simulink model "Evaluation_RL_SMC_Env"  (R2024b)
settings: Solver=VariableStepAuto  StartTime=0.0  StopTime=60  RelTol=1e-3
values from neighbouring files (symbols this model uses):
  D = [0; 0]    [K_vector_2.m]
undefined symbols (not defined in the file or in its folder): ref_seed
libraries: simulink x7, dspstat3 x4, rllib x2, slctrl_smc x1
settings Model: Creator=minhh  LastModifiedBy=minhh
settings DebuggingCC: SignalInfNanChecking=error

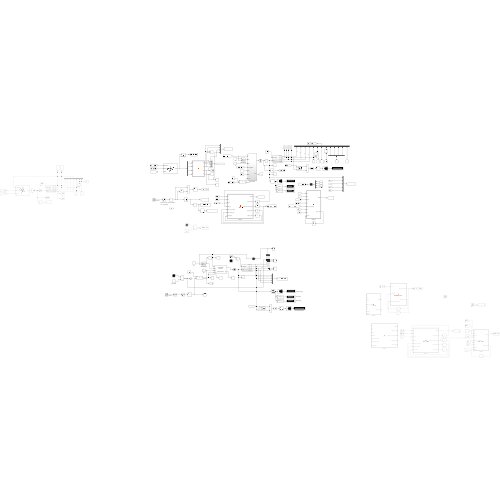
[thumbnail: Simulink's stored preview of the top-level diagram]
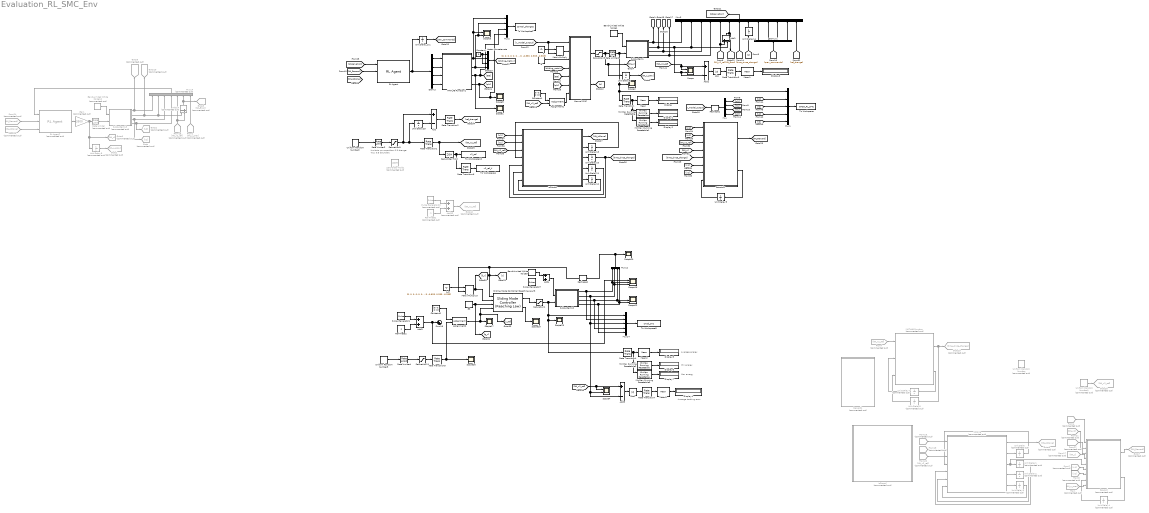
== system Evaluation_RL_SMC_Env ==
  note: Average energy
  note: Limits to no more than 0.3 change;
      | -0.2; 0.5 boundary
  note: Min energy
  note: Max energy
  note: Average tracking error
  A : Constant  Value=[0, 0, 0, 0; 0, 0, 0, 1; -4, 1, -0.5, 0.4; 0.833, -0.833, 0.333, -0.333]  VectorParams1D=off
  A_3 : Constant  Value=[0, 0, 0, 0; 0, 0, 0, 1; -4, 1, -0.5, 0.4; 0.833, -0.833, 0.333, -0.333]  VectorParams1D=off
  Abs : Abs  SaturateOnIntegerOverflow=off
  Abs1 : Abs  SaturateOnIntegerOverflow=off
  Add{,1..2,5} (4 alike) : Sum  Inputs=+-
  Add12 : Sum  Commented=on
  Add14 : Sum  Commented=on  Inputs=-+
  Add3 : Sum
  Add4 : Sum
  Assignment1 : Assignment  DiagnosticForDimensions=Warning  IndexOptions=Index vector (dialog)  Indices=2  OutputSizes=1
  Assignment2 : Assignment  DiagnosticForDimensions=Warning  IndexOptions=Index vector (dialog)  Indices=2  OutputSizes=1
  B : Constant  Value=[0; 0.004; 0; 0]
  B3 : Constant  Value=[0; 0.004; 0; 0]
  Band-Limited White Noise1 : simulink/Sources/Band-Limited White Noise  Cov=[200]  Ts=0.01  seed=23341
  Band-Limited White Noise12 : simulink/Sources/Band-Limited White Noise  Commented=on  Cov=[200]  Ts=0.01  seed=noise_seed
  Band-Limited White Noise9 : simulink/Sources/Band-Limited White Noise  Cov=[200]  Ts=0.01  seed=[23341]
  Constant : Constant  Value=0
  Constant1 : Constant  Value=[0; 0; 0; 0]  VectorParams1D=off
  Constant2 : Constant  Value=[0; 0; 0; 0]  VectorParams1D=off
  Demux : Demux
  Demux1 : Demux
  Display{,1..7} (8 alike) : Display
  From : From  Commented=on  GotoTag=NN_u_prev
  From1 : From  Commented=on  GotoTag=NN_u_prev
  From{7,15,20,22} (4 alike) : From  Commented=on  GotoTag=NN_x2_ref
  From17 : From  Commented=on  GotoTag=NN_u
  From18 : From  Commented=on  GotoTag=NN_x1
  From19 : From  Commented=on  GotoTag=NN_x2
  From2 : From  Commented=on  GotoTag=v1
  From21 : From  Commented=on  GotoTag=NN_x2
  From23 : From  Commented=on  GotoTag=NN_IsDone
  From24 : From  Commented=on  GotoTag=NN_Reward
  From3 : From  Commented=on  GotoTag=v2
  From4 : From  Commented=on  GotoTag=NN_x1
  Gain : Gain  Commented=on  Gain=3500
  Goto : Goto  Commented=on  GotoTag=v1
  Goto1 : Goto  Commented=on  GotoTag=NN_u_prev
  Goto10 : Goto  Commented=on  GotoTag=NN_x2
  Goto11 : Goto  Commented=on  GotoTag=NN_x2_ref
  Goto19 : Goto  Commented=on  GotoTag=time_since_change
  Goto2 : Goto  Commented=on  GotoTag=v2
  Goto28 : Goto  Commented=on  GotoTag=NN_x2_ref
  Goto5 : Goto  Commented=on  GotoTag=NN_Error
  Goto6 : Goto  Commented=on  GotoTag=NN_u
  Goto7 : Goto  Commented=on  GotoTag=NN_Reward
  Goto8 : Goto  Commented=on  GotoTag=NN_IsDone
  Goto9 : Goto  Commented=on  GotoTag=NN_x1
  IsDone : MATLAB Function  Commented=on  TreatAsAtomicUnit=on
  IsDone1 : MATLAB Function  Commented=on  TreatAsAtomicUnit=on
  IsDone2 : MATLAB Function  TreatAsAtomicUnit=on
  MATLAB Function : MATLAB Function  Commented=on  TreatAsAtomicUnit=on
  MATLAB Function1 : MATLAB Function  TreatAsAtomicUnit=on
  Manual SMC : Subsystem
  MatrixMultiply : Product  Multiplication=Matrix(*)
  MatrixMultiply3 : Product  Multiplication=Matrix(*)
  Mean{,1..3} (4 alike) : dspstat3/Mean  run=on  InputProcessing=Columns as channels (frame based)  reset_popup=None  directionMode=Each column  dimension=1  roiEnable=off  roiType=Rectangles  roiPortion=Entire ROI  roiOutput=Individual statistics for each ROI  roiFlag=off  roundingMode=Floor  overflowMode=off  outputDataTypeStr=Inherit: Same as accumulator  outputMin=[]  outputMax=[]  outputLastDataTypeStr=Inherit: Same as accumulator
  MinMax Running Resettable : simulink/Math Operations/MinMax Running Resettable  Function=min  vinit=0.0
  MinMax Running Resettable1 : simulink/Math Operations/MinMax Running Resettable  Function=max  vinit=0.0
  MinMax Running Resettable2 : simulink/Math Operations/MinMax Running Resettable  Function=min  vinit=0.0
  MinMax Running Resettable3 : simulink/Math Operations/MinMax Running Resettable  Function=max  vinit=0.0
  Mux : Mux
  Mux1 : Mux  Inputs=5
  Mux12 : Mux
  Mux14 : Mux  Inputs=5
  Mux19 : Mux  Commented=on  Inputs=7
  Mux2 : Mux
  Mux3 : Mux  Inputs=13
  Pulse Generator1 : DiscretePulseGenerator  PulseType=Time based  Amplitude=0.3  Period=100  PulseWidth=20  PhaseDelay=20
  Pulse Generator10 : DiscretePulseGenerator  Commented=on  PulseType=Time based  Amplitude=0.3  Period=100  PulseWidth=20  PhaseDelay=20
  Pulse Generator7 : DiscretePulseGenerator  PulseType=Time based  Amplitude=500  Period=100  PulseWidth=.1
  RL Agent : rllib/RL Agent  Agent=metaObj_ep_3971  ExternalActionAsInput=off  ProvideLastAction=off  ProvideCumRwd=off  TreatAsDirectFeedthrough=on  UseStrictObservationDataTypes=off
  RL Agent2 : rllib/RL Agent  Commented=on  Agent=agentObj  ExternalActionAsInput=off  ProvideLastAction=off  ProvideCumRwd=off  TreatAsDirectFeedthrough=on  UseStrictObservationDataTypes=off
  Rate Limiter : RateLimiter  Commented=on  RisingSlewLimit=25000  FallingSlewLimit=-25000  SampleTimeMode=inherited
  Rate Limiter1 : RateLimiter  RisingSlewLimit=25000  FallingSlewLimit=-25000  SampleTimeMode=inherited
  Rate Limiter2 : RateLimiter  RisingSlewLimit=0.1  FallingSlewLimit=-0.1  SampleTimeMode=inherited
  Rate Limiter4 : RateLimiter  RisingSlewLimit=0.1  FallingSlewLimit=-0.1  SampleTimeMode=inherited
  Rate Transition{,1..5,7} (7 alike) : RateTransition  OutPortSampleTime=0.01
  Rate Transition6 : RateTransition  OutPortSampleTime=0.02
  Ref Theta1 : Constant  Commented=on  Value=.1
  Ref Theta2 : Constant  Value=.1
  Reshape1 : Reshape  OutputDimensionality=Column vector (2-D)
  Reshape2 : Reshape  OutputDimensionality=Column vector (2-D)
  Reward : MATLAB Function  Commented=on  TreatAsAtomicUnit=on
  Reward1 : MATLAB Function  Commented=on  TreatAsAtomicUnit=on
  Reward2 : MATLAB Function  TreatAsAtomicUnit=on
  Saturation1 : Saturate  UpperLimit=3500  LowerLimit=-3500
  Saturation11 : Saturate  LowerLimit=-0.2
  Saturation8 : Saturate  UpperLimit=3500  LowerLimit=-3500
  Saturation9 : Saturate  LowerLimit=-0.2
  Scope : Scope  NumInputPorts=2
  Scope{1..2,5,17,19..20,23,26} (8 alike) : Scope
  Scope16 : Scope  NumInputPorts=3
  Scope22 : Scope  NumInputPorts=3
  Scope3 : Scope  NumInputPorts=2
  Scope4 : Scope  NumInputPorts=2
  Sliding Mode Controller (Reaching Law)3 : slctrl_smc/Sliding Mode Controller (Reaching Law)  TaskMode=Tracking Mode  SlidingMatrix=[0; 15; 0; 2]  EnableTrackingDerivative=off  EnableSwitchingFunction=on  ReachingLaw=Exponential  ReachingRate=100  ControlGain=10  PowerRate=1  BoundaryLayer=Hyperbolic Tangent  ZeroCross=off  Phi=0.1
  Subsystem1 : Subsystem
  Subsystem10 : Subsystem
  Subsystem13 : Subsystem  Commented=on
  Sum18 : Sum  Inputs=|++
  To Workspace : ToWorkspace  VariableName=CMSD_RL_SMC  SaveFormat=Timeseries  SampleTime=-1
  To Workspace1 : ToWorkspace  VariableName=x2_ref_rl  SampleTime=-1
  To Workspace10 : ToWorkspace  VariableName=x2_ref  SampleTime=-1
  To Workspace2 : ToWorkspace  VariableName=control_changes  SaveFormat=Timeseries  SampleTime=-1
  To Workspace8 : ToWorkspace  VariableName=cmsd_smc  SampleTime=0.1
  Uniform Random Number : UniformRandomNumber  Commented=on  Minimum=0  Maximum=0.5  Seed=ref_seed  SampleTime=10
  Uniform Random Number1 : UniformRandomNumber  Commented=on  Minimum=-0.2  Maximum=0.5  Seed=12311  SampleTime=3
  Uniform Random Number2 : UniformRandomNumber  Minimum=-0.2  Maximum=0.5  Seed=12345  SampleTime=3
  Uniform Random Number3 : UniformRandomNumber  Minimum=-0.2  Maximum=0.5  Seed=12345  SampleTime=3
  Unit Delay{,1..5,7} (7 alike) : UnitDelay  Commented=on  SampleTime=0.01  HasFrameUpgradeWarning=on
  Unit Delay{6,9..13} (6 alike) : UnitDelay  SampleTime=0.01  HasFrameUpgradeWarning=on
  Unit Delay14 : UnitDelay  SampleTime=-1  HasFrameUpgradeWarning=on
  Unit Delay25 : UnitDelay  SampleTime=3  HasFrameUpgradeWarning=on
  Unit Delay8 : UnitDelay  Commented=on  InitialCondition=0.0  SampleTime=0.01  HasFrameUpgradeWarning=on
  Unit Delay_0.1 : UnitDelay  InitialCondition=[0; 0; 0; 0]  SampleTime=0.1  HasFrameUpgradeWarning=on
  Vector Concatenate : Concatenate  NumInputs=4
  Zero-Order Hold : ZeroOrderHold  SampleTime=0.1
  Zero-Order Hold1 : ZeroOrderHold  Commented=on  SampleTime=0.1
  wires:
  From20/1 -> IsDone/3(x2_ref)
  IsDone/5(next_ref_prev) -> Unit Delay3/1
  Unit Delay/1 -> IsDone/4(timer_03)
  From22/1 -> Reward/3(x2_ref)
  IsDone/2(next_timer_03) -> Unit Delay/1
  Unit Delay1/1 -> IsDone/5(time_since_change)
  From18/1 -> IsDone/1(x1)
  Unit Delay2/1 -> IsDone/6(current_step_size)
  From19/1 -> IsDone/2(x2)
  Add14/1 -> Goto5/1, Mux19/6
  Reward/2(next_x2_prev) -> Unit Delay4/1
  Unit Delay3/1 -> IsDone/7(x2_ref_prev)
  From17/1 -> Reward/4(u)
  From24/1 -> RL Agent2/2
  Unit Delay4/1 -> Reward/8(x2_prev)
  Rate Limiter/1 -> Subsystem13/2(u (N))
  IsDone/4(next_step_size) -> Unit Delay2/1
  From15/1 -> Mux19/5, Add14/2
  IsDone/1(is_done) -> Goto8/1
  Band-Limited White Noise12/1 -> Subsystem13/1(disturbance)
  Reward/1(reward) -> Goto7/1
  Subsystem13/4(Vel_2) -> Goto2/1, Mux19/4  "v2"
  From21/1 -> Reward/2(x2)
  Subsystem13/1(Pos_1) -> Mux19/1, Goto9/1  "x1"
  From23/1 -> RL Agent2/3
  Subsystem13/2(Pos_2) -> Add14/1, Mux19/2, Goto10/1  "x2"
  IsDone/3(next_time_since_change) -> Reward/5(time_since_change), Unit Delay1/1
  Subsystem13/3(Vel_1) -> Goto/1, Mux19/3  "v1"
  RL Agent2/1 -> Gain/1
  From/1 -> Reward/9(u_prev)
  Gain/1 -> Unit Delay5/1, Goto6/1, Rate Limiter/1
  Unit Delay5/1 -> Goto1/1
  From1/1 -> Mux19/7
  Mux19/1 -> RL Agent2/1
  From2/1 -> Reward/6(v1)
  From3/1 -> Reward/7(v2)
  From4/1 -> Reward/1(x1)
  Band-Limited White Noise1/1 -> Subsystem1/1(disturbance)
  Rate Limiter1/1 -> Mux1/1, Rate Transition/1, Scope2/1, Subsystem1/2(u (N))
  Manual SMC/1(u) -> Saturation8/1
  Unit Delay6/1 -> [NN_u_prev]
  Manual SMC/2(Slope) -> [s]
  Subsystem1/1(Pos_1) -> Mux3/1, [x1]  "x1"
  Subsystem1/2(Pos_2) -> Add2/2, Scope/2, Mux3/2, Add1/2, [x2]  "x2"
  Subsystem1/3(Vel_1) -> Mux3/3, [v1]  "v1"
  Add1/1 -> [NN_Error], Mux3/6
  Subsystem1/4(Vel_2) -> Mux3/4, [v2]  "x2"
  [NN_x2_ref] -> Mux3/5, Add1/1
  RL Agent/1 -> Unit Delay_0.1/1, Demux/1
  [x1] -> Mux/1
  [x2] -> Mux/2
  [v1] -> Mux/3
  [v2] -> Mux/4
  Mux/1 -> Reshape1/1
  Reshape1/1 -> [x_model_output]
  [x_model_output] -> MatrixMultiply/2, Manual SMC/1(x)
  A/1 -> MatrixMultiply/1
  MatrixMultiply/1 -> Manual SMC/2(f(x))
  B/1 -> Manual SMC/3(g(x))
  [NN_x2_ref] -> Assignment1/2
  Constant1/1 -> Assignment1/1
  Assignment1/1 -> Manual SMC/7(x_ref)  "Reference"
  MATLAB Function/2(next_x2_ref_prev) -> Unit Delay7/1
  Unit Delay7/1 -> MATLAB Function/2(x2_ref_prev)
  MATLAB Function/1(time_since_change) -> Goto19/1, Unit Delay8/1
  Unit Delay8/1 -> MATLAB Function/3(time_since_change_prev)
  From7/1 -> MATLAB Function/1(x2_ref)
  [time_since_change] -> Mux3/7
  [s] -> Unit Delay14/1
  Unit Delay_0.1/1 -> [prev_commands]
  Demux1/4 -> Mux3/12
  Demux1/3 -> Mux3/11
  Demux1/2 -> Mux3/10
  Demux1/1 -> Mux3/9
  [prev_commands] -> Demux1/1
  Mux3/1 -> [observation]
  [observation] -> RL Agent/1
  Constant/1 -> Vector Concatenate/3, Vector Concatenate/1
  Vector Concatenate/1 -> [sliding_matrix]
  [sliding_matrix] -> Manual SMC/4(Sliding Matrix)
  [eta] -> Manual SMC/5(Eta)
  [phi] -> Manual SMC/6(Phi)
  Demux/1 -> MATLAB Function1/1(u1)
  Demux/2 -> MATLAB Function1/2(u2)
  Demux/3 -> MATLAB Function1/3(u3)
  Demux/4 -> MATLAB Function1/4(u4)
  MATLAB Function1/1(C2) -> Mux2/1, Scope3/1, Vector Concatenate/2
  MATLAB Function1/2(C4) -> Mux2/2, Scope3/2, Vector Concatenate/4
  MATLAB Function1/3(Eta) -> Mux2/3, [eta], Scope1/1
  MATLAB Function1/4(Phi) -> Mux2/4, Scope5/1, [phi]
  Reward2/1(reward) -> [NN_Reward]
  Reward2/2(next_u_prev) -> Unit Delay9/1
  Unit Delay9/1 -> Reward2/8(u_prev)
  [time_since_change] -> Reward2/5(time_since_change)
  [v1] -> Reward2/6(v1)
  Saturation8/1 -> Unit Delay6/1, [NN_u], Rate Limiter1/1
  [NN_u] -> Reward2/4(u)
  [NN_x2_ref] -> Reward2/3(x2_ref)
  [x2] -> Reward2/2(x2)
  [x1] -> Reward2/1(x1)
  [v2] -> Reward2/7(v2)
  IsDone2/3(next_time_since_change) -> Unit Delay10/1
  IsDone2/4(next_step_size) -> Unit Delay11/1
  IsDone2/5(next_ref_prev) -> Unit Delay12/1
  Unit Delay12/1 -> IsDone2/7(x2_ref_prev)
  Unit Delay11/1 -> IsDone2/6(current_step_size)
  Unit Delay10/1 -> [time_since_change], IsDone2/5(time_since_change)
  IsDone2/1(is_done) -> [NN_IsDone]
  IsDone2/2(next_timer_03) -> Unit Delay13/1
  Unit Delay13/1 -> IsDone2/4(timer_03)
  [x1] -> IsDone2/1(x1)
  [x2] -> IsDone2/2(x2)
  [NN_x2_ref] -> IsDone2/3(x2_ref)
  Unit Delay14/1 -> Mux3/8
  [NN_Reward] -> RL Agent/2
  Ref Theta1/1 -> Add12/2
  Pulse Generator10/1 -> Add12/1
  Add12/1 -> Goto11/1  "Reference"
  Mean/1 -> Display/1
  Rate Transition/1 -> MinMax Running Resettable1/1, MinMax Running Resettable/1, Mean/1
  MinMax Running Resettable/1 -> Display1/1
  MinMax Running Resettable1/1 -> Display2/1
  Uniform Random Number1/1 -> Goto28/1  "Reference"
  Uniform Random Number2/1 -> Rate Limiter2/1  "Reference"
  Saturation9/1 -> Add/1, Unit Delay25/1, Rate Transition1/1
  Add/1 -> Rate Transition2/1
  Rate Transition2/1 -> [ref_change]
  Rate Limiter2/1 -> Saturation9/1
  Unit Delay25/1 -> Add/2
  [ref_change] -> Mux3/13
  [NN_x2_ref] -> Add2/1, Scope/1
  Add2/1 -> Abs/1
  Rate Transition3/1 -> Mean1/1
  Mean1/1 -> Display3/1
  Abs/1 -> Rate Transition3/1
  Mux1/1 -> To Workspace/1
  [x1] -> Mux1/2
  [x2] -> Mux1/3
  [v1] -> Mux1/4
  [v2] -> Mux1/5
  MinMax Running Resettable2/1 -> Display6/1
  Mean2/1 -> Display5/1
  MinMax Running Resettable3/1 -> Display7/1
  Rate Transition4/1 -> MinMax Running Resettable3/1, MinMax Running Resettable2/1, Mean2/1
  A_3/1 -> MatrixMultiply3/1
  Subsystem10/4(Vel_2) -> Scope22/3, Mux12/4, Mux14/5  "v2"
  Add4/1 -> Subsystem10/1(disturbance)
  Uniform Random Number3/1 -> Rate Limiter4/1  "Reference"
  Rate Limiter4/1 -> Saturation11/1
  Band-Limited White Noise9/1 -> Add4/1
  Subsystem10/3(Vel_1) -> Mux14/4, Scope22/2, Mux12/3  "v1"
  Mux14/1 -> To Workspace8/1
  Saturation11/1 -> Rate Transition5/1
  Sliding Mode Controller (Reaching Law)3/2 -> Scope19/1
  MatrixMultiply3/1 -> [f_x], Sliding Mode Controller (Reaching Law)3/2
  Rate Transition5/1 -> Scope26/1, Assignment2/2
  Pulse Generator1/1 -> Add3/1
  Subsystem10/1(Pos_1) -> Mux14/2, Scope16/2, Mux12/1  "x1"
  Constant2/1 -> Assignment2/1
  Mux12/1 -> Scope20/1, Reshape2/1
  B3/1 -> [g_x], Sliding Mode Controller (Reaching Law)3/3
  Ref Theta2/1 -> Add3/2
  Saturation1/1 -> Subsystem10/2(u (N)), Rate Transition4/1, Scope23/1, Mux14/1  "u"
  Reshape2/1 -> MatrixMultiply3/2, [x], Sliding Mode Controller (Reaching Law)3/1
  Assignment2/1 -> [x_ref], Sliding Mode Controller (Reaching Law)3/4, Scope17/1  "Reference"
  Sliding Mode Controller (Reaching Law)3/1 -> Saturation1/1
  Add3/1 -> Scope16/1, Sum18/1  "Reference"
  Rate Transition1/1 -> Zero-Order Hold/1, [NN_x2_ref]
  Zero-Order Hold/1 -> Rate Transition6/1, To Workspace10/1
  Rate Transition6/1 -> To Workspace1/1
  Add5/1 -> Abs1/1
  Rate Transition7/1 -> Mean3/1
  Abs1/1 -> Rate Transition7/1
  [NN_x2_ref] -> Add5/1, Scope4/1
  Subsystem10/2(Pos_2) -> Scope4/2, Add5/2, Mux14/3, Scope16/3, Mux12/2  "x2"
  Mean3/1 -> Display4/1
  Mux2/1 -> To Workspace2/1

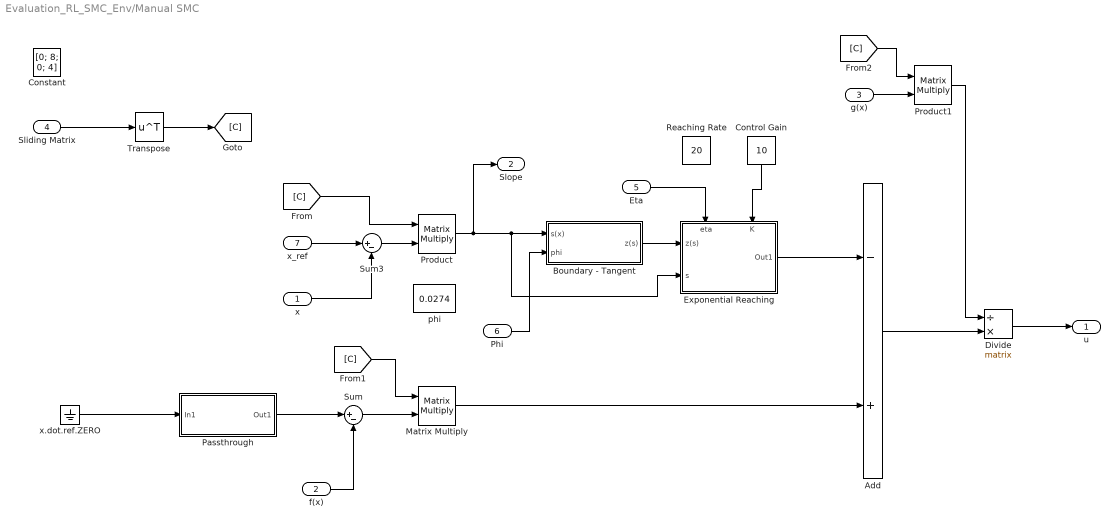
== system Evaluation_RL_SMC_Env/Manual SMC ==
  x : Inport
  f(x) : Inport  Port=2
  g(x) : Inport  Port=3
  Sliding Matrix : Inport  Port=4
  Eta : Inport  Port=5
  Phi : Inport  Port=6
  x_ref : Inport  Port=7
  Add : Sum  Inputs=-+
  Boundary - Tangent : Subsystem
  Constant : Constant  Value=[0; 8; 0; 4]  VectorParams1D=off
  Control Gain : Constant  Value=10
  Divide : Product  Inputs=/*  Multiplication=Matrix(*)
  Exponential Reaching : Subsystem
      settings: PortSchema="{\"entries\":[{\"content\":{\"sides\":[{\"content\":{\"connectorIds\":[\"In1\",\"In2\"]},\"type\":\"ConnectorPlacement.EquallySpacedRectSide\",\"uuid\":\"14532932-ba42-4254-ad37-14ae2c40c086\"},{\"content\":{\"connectorIds\":[\"Out1\"],\"side\":\"RIGHT\"},\"type\":\"ConnectorPlacement.EquallySpacedRectSide\",\"uuid\":\"b67c1209-83dd-4fb0-99c8-05226babf43d\"},{\"content\":{\"connectorIds\":[\"In3\",\"In4\"],\"side\":\"TOP\"},\"type\":\"ConnectorPlacement.EquallySpacedRectSide\",\"uuid\":\"11cfd510-8790-4762-abc8-282610a147ed\"}]},\"type\":\"ConnectorPlacement.EquallySpacedConnector\",\"uuid\":\"c799e45e-6b6c-4526-9867-c33aadee095c\"}],\"packageUris\":[\"http://schema.mathworks.com/mf0/Connector/R2020b\"],\"version\":\"1.0\"}"
  Matrix Multiply : Product  Multiplication=Matrix(*)
  Passthrough : Subsystem  Variant=on
  Product : Product  Multiplication=Matrix(*)
  Product1 : Product  Multiplication=Matrix(*)
  Reaching Rate : Constant  Value=20
  Sum : Sum  Inputs=|+-
  Sum3 : Sum  Inputs=|+-
  Transpose : Math  Operator=transpose
  phi : Constant  Value=0.0274
  x.dot.ref.ZERO : Ground
  u : Outport
  Slope : Outport  Port=2
  wires:
  Transpose/1 -> [C]
  [C] -> Product/1
  x/1 -> Sum3/2
  x_ref/1 -> Sum3/1
  Sum3/1 -> Product/2
  x.dot.ref.ZERO/1 -> Passthrough/1(In1)
  Passthrough/1(Out1) -> Sum/1
  f(x)/1 -> Sum/2
  Sum/1 -> Matrix Multiply/2
  [C] -> Matrix Multiply/1
  Product/1 -> Slope/1, Exponential Reaching/2(s), Boundary - Tangent/1(s(x))
  Control Gain/1 -> Exponential Reaching/4(K)
  Boundary - Tangent/1(z(s)) -> Exponential Reaching/1(z(s))
  Exponential Reaching/1(Out1) -> Add/1
  Matrix Multiply/1 -> Add/2
  [C] -> Product1/1
  g(x)/1 -> Product1/2
  Add/1 -> Divide/2
  Product1/1 -> Divide/1
  Divide/1 -> u/1
  Sliding Matrix/1 -> Transpose/1
  Phi/1 -> Boundary - Tangent/2(phi)
  Eta/1 -> Exponential Reaching/3(eta)

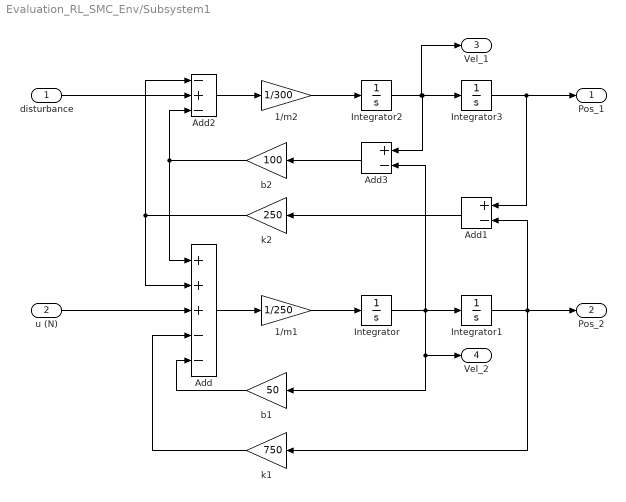
== system Evaluation_RL_SMC_Env/Subsystem1 ==
  disturbance : Inport
  u (N) : Inport  Port=2
  1/m1 : Gain  Gain=1/250
  1/m2 : Gain  Gain=1/300
  Add : Sum  Inputs=+++--
  Add1 : Sum  Inputs=+-
  Add2 : Sum  Inputs=-+-
  Add3 : Sum  Inputs=+-
  Integrator{,1..3} (4 alike) : Integrator
  b1 : Gain  Gain=50
  b2 : Gain  Gain=100
  k1 : Gain  Gain=750
  k2 : Gain  Gain=250
  Pos_1 : Outport
  Pos_2 : Outport  Port=2
  Vel_1 : Outport  Port=3
  Vel_2 : Outport  Port=4
  wires:
  Add/1 -> 1/m1/1
  1/m1/1 -> Integrator/1
  Integrator/1 -> Add3/2, Integrator1/1, b1/1, Vel_2/1
  Integrator1/1 -> k1/1, Pos_2/1, Add1/2
  Add2/1 -> 1/m2/1
  1/m2/1 -> Integrator2/1
  Integrator2/1 -> Vel_1/1, Add3/1, Integrator3/1
  Add3/1 -> b2/1
  b2/1 -> Add2/3, Add/1
  Add1/1 -> k2/1
  Integrator3/1 -> Pos_1/1, Add1/1
  u (N)/1 -> Add/3
  b1/1 -> Add/5
  k1/1 -> Add/4
  k2/1 -> Add2/1, Add/2
  disturbance/1 -> Add2/2

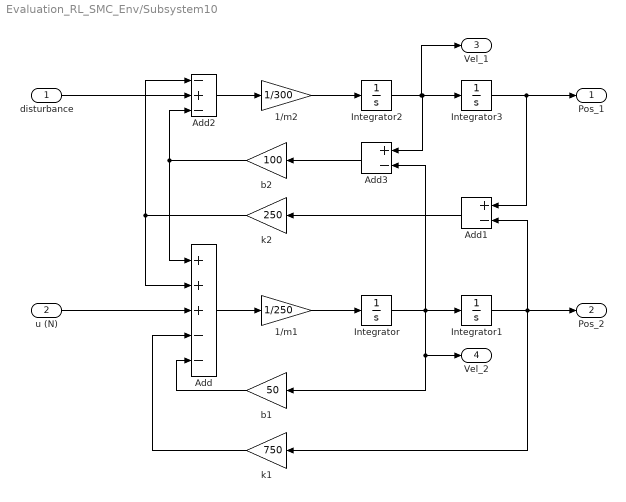
== system Evaluation_RL_SMC_Env/Subsystem10 ==
  disturbance : Inport
  u (N) : Inport  Port=2
  1/m1 : Gain  Gain=1/250
  1/m2 : Gain  Gain=1/300
  Add : Sum  Inputs=+++--
  Add1 : Sum  Inputs=+-
  Add2 : Sum  Inputs=-+-
  Add3 : Sum  Inputs=+-
  Integrator{,1..3} (4 alike) : Integrator
  b1 : Gain  Gain=50
  b2 : Gain  Gain=100
  k1 : Gain  Gain=750
  k2 : Gain  Gain=250
  Pos_1 : Outport
  Pos_2 : Outport  Port=2
  Vel_1 : Outport  Port=3
  Vel_2 : Outport  Port=4
  wires:
  Add/1 -> 1/m1/1
  1/m1/1 -> Integrator/1
  Integrator/1 -> Add3/2, Integrator1/1, b1/1, Vel_2/1
  Integrator1/1 -> k1/1, Pos_2/1, Add1/2
  Add2/1 -> 1/m2/1
  1/m2/1 -> Integrator2/1
  Integrator2/1 -> Vel_1/1, Add3/1, Integrator3/1
  Add3/1 -> b2/1
  b2/1 -> Add2/3, Add/1
  Add1/1 -> k2/1
  Integrator3/1 -> Pos_1/1, Add1/1
  u (N)/1 -> Add/3
  b1/1 -> Add/5
  k1/1 -> Add/4
  k2/1 -> Add2/1, Add/2
  disturbance/1 -> Add2/2

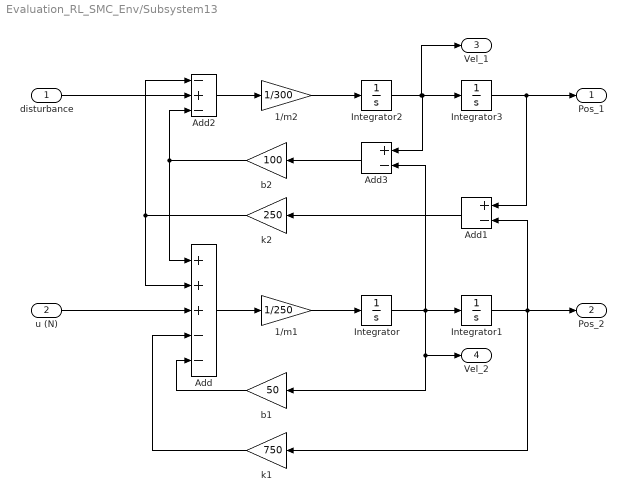
== system Evaluation_RL_SMC_Env/Subsystem13 ==
  disturbance : Inport
  u (N) : Inport  Port=2
  1/m1 : Gain  Gain=1/250
  1/m2 : Gain  Gain=1/300
  Add : Sum  Inputs=+++--
  Add1 : Sum  Inputs=+-
  Add2 : Sum  Inputs=-+-
  Add3 : Sum  Inputs=+-
  Integrator{,1..3} (4 alike) : Integrator
  b1 : Gain  Gain=50
  b2 : Gain  Gain=100
  k1 : Gain  Gain=750
  k2 : Gain  Gain=250
  Pos_1 : Outport
  Pos_2 : Outport  Port=2
  Vel_1 : Outport  Port=3
  Vel_2 : Outport  Port=4
  wires:
  Add/1 -> 1/m1/1
  1/m1/1 -> Integrator/1
  Integrator/1 -> Add3/2, Integrator1/1, b1/1, Vel_2/1
  Integrator1/1 -> k1/1, Pos_2/1, Add1/2
  Add2/1 -> 1/m2/1
  1/m2/1 -> Integrator2/1
  Integrator2/1 -> Vel_1/1, Add3/1, Integrator3/1
  Add3/1 -> b2/1
  b2/1 -> Add2/3, Add/1
  Add1/1 -> k2/1
  Integrator3/1 -> Pos_1/1, Add1/1
  u (N)/1 -> Add/3
  b1/1 -> Add/5
  k1/1 -> Add/4
  k2/1 -> Add2/1, Add/2
  disturbance/1 -> Add2/2

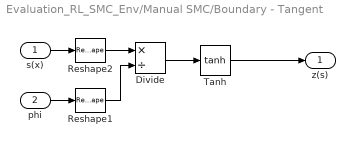
== system Evaluation_RL_SMC_Env/Manual SMC/Boundary - Tangent ==
  s(x) : Inport
  phi : Inport  Port=2
  Divide : Product  Inputs=*/
  Reshape1 : Reshape  OutputDimensionality=Column vector (2-D)
  Reshape2 : Reshape  OutputDimensionality=Column vector (2-D)
  Tanh : Trigonometry  Operator=tanh
  z(s) : Outport
  wires:
  Reshape1/1 -> Divide/2
  Divide/1 -> Tanh/1
  phi/1 -> Reshape1/1
  Reshape2/1 -> Divide/1
  Tanh/1 -> z(s)/1
  s(x)/1 -> Reshape2/1

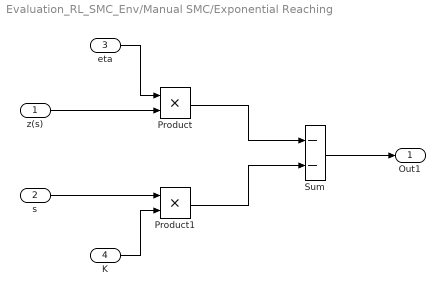
== system Evaluation_RL_SMC_Env/Manual SMC/Exponential Reaching ==
  z(s) : Inport
  s : Inport  Port=2
  eta : Inport  Port=3
  K : Inport  Port=4
  Product : Product  Inputs=**
  Product1 : Product
  Sum : Sum  Inputs=--
  Out1 : Outport
  wires:
  z(s)/1 -> Product/2
  eta/1 -> Product/1
  s/1 -> Product1/1
  K/1 -> Product1/2
  Product/1 -> Sum/1
  Product1/1 -> Sum/2
  Sum/1 -> Out1/1

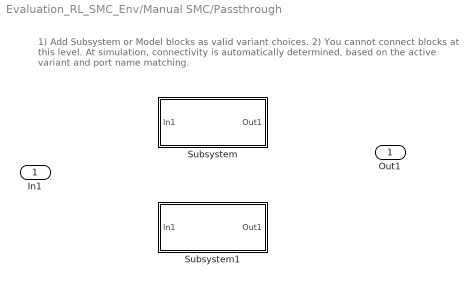
== system Evaluation_RL_SMC_Env/Manual SMC/Passthrough ==
  note: 1) Add Subsystem or Model blocks as valid variant choices.
      | 2) You cannot connect blocks at this level. At simulation, connectivity is automatically
      | determined, based on the active variant and port name matching.
  In1 : Inport
  Subsystem : Subsystem  VariantControl=true
  Subsystem1 : Subsystem  VariantControl=false
  Out1 : Outport

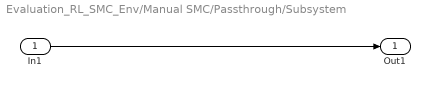
== system Evaluation_RL_SMC_Env/Manual SMC/Passthrough/Subsystem ==
  In1 : Inport
  Out1 : Outport
  wires:
  In1/1 -> Out1/1

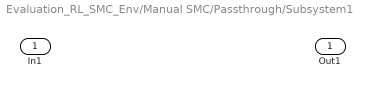
== system Evaluation_RL_SMC_Env/Manual SMC/Passthrough/Subsystem1 ==
  In1 : Inport
  Out1 : Outport

== matlab function Evaluation_RL_SMC_Env/Reward ==
  data: x1 input; x2 input; x2_ref input; u input; time_since_change input; v1 input; v2 input; reward output; x2_prev input; next_x2_prev output; u_prev input
function [reward, next_x2_prev] = calc_reward(x1, x2, x2_ref, u, time_since_change, v1, v2, x2_prev, u_prev)

% =========================================================================
% calc_reward.m — CMSD NN Controller Reward Function (v5)
%
% Root cause fix: dying fast was more profitable than surviving.
% Per-step cost (-2.48) exceeded per-step income (+0.1) when tracking
% was poor, so the agent rationally chose quick death over long survival.
%
% Fix: base reward raised to +1.0, progress bonus widened so it pays out
% even at 0.3m error, miss penalties removed (quadratic handles distance).
% Now every step alive is net positive, tracking well is 7x better than
% tracking poorly, and dying is always worse than surviving.
%
% Per-step economics (v5):
%   Poor tracking (error=0.3m): +1.0 + 0.64 - 0.9 = +0.74/step (net positive)
%   Good tracking (error=0.01m): +1.0 + 1.0 + 3.0 - 0.001 = +4.99/step
%   Perfect tracking (error=0):  +5.0/step
%   6000-step perfect episode:   ~+30,000 total
% =========================================================================

% --- DATA TYPES ---
    reward       = double(1.0);           % raised from 0.1 — survival has inherent value
    next_x2_prev = double(x2);
    x2_error     = double(abs(x2_ref - x2));
    delta_u      = double(abs(u - u_prev));
    x1_abs       = double(abs(x1));

% --- 1. TRACKING — primary goal ---
%   Quadratic penalty. At error=0.3m: -0.9. At error=1.0m: -10.
%   Kept unchanged — this is the core learning signal.
    reward = double(reward - (10.0 * x2_error^2));

% --- 2. ZONE BONUS (penalties removed) ---
%   Previous version penalised being far from target on top of the
%   quadratic. This double-penalised poor tracking and made per-step cost
%   exceed per-step income, incentivising fast death.
%   Now: bonuses only. Being far costs only through the quadratic term.
    if x2_error < 0.010
        reward = double(reward + 3.0);    % inside 10mm  — excellent
    elseif x2_error < 0.050
        reward = double(reward + 1.5);    % inside 50mm  — good
    elseif x2_error < 0.150
        reward = double(reward + 0.3);    % inside 150mm — acceptable, small bonus
    % No penalty beyond 150mm — quadratic term handles it
    end

% --- 3. PROGRESS / SURVIVAL BONUS ---
%   Widened Gaussian (sigma doubled: -20 -> -5) so bonus pays even at 0.3m.
%   This is what makes every step alive net positive regardless of tracking.
%   At error=0.0m:  +1.0/step (excellent, doubles the base survival reward)
%   At error=0.1m:  +0.95/step (still very good)
%   At error=0.3m:  +0.64/step (meaningful — agent wants to stay alive)
%   At error=1.0m:  +0.007/step (essentially zero — must track to benefit)
    progress_bonus = double(1.0 * exp(-5.0 * x2_error^2));
    reward = double(reward + progress_bonus);

% --- 4. VELOCITY DAMPING after settling ---
%   Only after 1s grace period following reference change.
    if time_since_change > 1.0
        if abs(v2) > 0.05
            reward = double(reward - 1.0);
        end
        if abs(v1) > 0.05
            reward = double(reward - 0.5);
        end
    end

% --- 5. ENERGY EFFICIENCY ---
%   Very small — tiebreaker only, does not dominate learning signal.
    reward = double(reward - 0.01 * (u / 3500.0)^2);

% --- 6. HARDWARE JERK PENALTY — LINEAR ---
    if delta_u > 500.0
        violation = double(delta_u - 500.0);
        reward    = double(reward - (0.005 * violation));
    end

% --- 7. X1 SOFT BARRIER ---
%   Zone-1 from 0.30m, Zone-2 from 0.45m.
%   At x1=0.65m: total ~-1.46/step — costly but not overwhelming.
%   Terminal -500 makes wall approach unambiguously fatal.
    if x1_abs > 0.30
        x1_margin1 = double(x1_abs - 0.30);
        reward = double(reward - (8.0 * x1_margin1^2));
    end
    if x1_abs > 0.45
        x1_margin2 = double(x1_abs - 0.45);
        reward = double(reward - (12.0 * x1_margin2^2));
    end

% --- 8. X1 CENTERING BONUS ---
%   Continuous pull toward x1=0. +0.30/step at centre, fades beyond 0.40m.
    x1_centre_bonus = double(0.30 * exp(-10.0 * x1^2));
    reward = double(reward + x1_centre_bonus);

% --- 9. X1 TERMINAL PENALTY ---
    if x1_abs > 0.65
        reward = double(reward - 500.0);
    end

% --- 10. PER-STEP HARD FLOOR ---
%   Still needed for jerk/barrier spikes. -50 allows large penalties
%   without gradient-destroying billion-scale values.
    reward = double(max(reward, -50.0));

end

== matlab function Evaluation_RL_SMC_Env/IsDone ==
  data: x1 input; is_done output; x2 input; x2_ref input; next_timer_03 output; timer_03 input; time_since_change input; current_step_size input; x2_ref_prev input; next_time_since_change output; next_step_size output; next_ref_prev output
function [is_done, next_timer_03, next_time_since_change, next_step_size, next_ref_prev] = check_safety(x1, x2, x2_ref, timer_03, time_since_change, current_step_size, x2_ref_prev)

% =========================================================================
% check_safety.m — CMSD Episode Termination (v2)
%
% Changes from v1:
%   - Settle timeout is now PROPORTIONAL to step size (was flat 8.0s)
%     Flat 8s allowed the agent to idle on small steps, contributing to
%     the "do nothing and survive" local minimum seen at episode 150.
%   - x2 error timer threshold widened to 0.5m (kept from v1)
%   - All fprintf diagnostics kept — remove when no longer needed
% =========================================================================

% --- DATA TYPES ---
    is_done                = double(0);
    next_timer_03          = double(timer_03);
    next_time_since_change = double(time_since_change);
    next_step_size         = double(current_step_size);
    next_ref_prev          = double(x2_ref_prev);
    dt                     = double(0.01);
    x2_error               = double(x2_ref - x2);

% --- 1. REFERENCE CHANGE DETECTION ---
    if abs(x2_ref - x2_ref_prev) > 0.001
        next_time_since_change = double(0.0);
        next_step_size         = double(abs(x2_ref - x2_ref_prev));
    else
        next_time_since_change = double(time_since_change + dt);
    end
    next_ref_prev = double(x2_ref);

% --- 2. DEATH A: x1 hard wall ---
    if abs(x1) > 0.65
        is_done = double(1);
        fprintf('DEATH: x1 wall at x1=%.3f\n', x1);
    end

% --- 3. DEATH B: x2 error timer ---
%   Threshold 0.5m — wide enough that normal transients don't trigger it.
%   3 second timer — recycles a completely lost agent quickly.
    error_threshold = double(0.5);
    timer_duration  = double(3.0);

    if abs(x2_error) > error_threshold
        next_timer_03 = double(timer_03 + dt);
    else
        next_timer_03 = double(0.0);
    end

    if next_timer_03 > timer_duration
        is_done = double(1);
        fprintf('DEATH: x2 error timer at x2_err=%.3f\n', abs(x2_error));
    end

% --- 4. DEATH C: settle-time (PROPORTIONAL to step size) ---
%   Flat 8.0s was allowing the agent to idle on small reference steps.
%   A 0.05m step should settle in ~2s. A 1.5m step may need 6s.
%   Formula: max(3.0s minimum, step_size * 4.0 seconds/metre)
%   Examples:
%     step = 0.10m  →  allowed = max(3.0, 0.40) = 3.0s
%     step = 0.50m  →  allowed = max(3.0, 2.00) = 3.0s
%     step = 0.80m  →  allowed = max(3.0, 3.20) = 3.2s
%     step = 1.50m  →  allowed = max(3.0, 6.00) = 6.0s
%   Error band: 50mm — tighten to 30mm once agent survives 1000+ steps
    if next_step_size > 0
        allowed_settle_time = double(max(3.0, next_step_size * 4.0));
    else
        allowed_settle_time = double(3.0);
    end
    error_band = double(0.050);

    if (next_time_since_change > allowed_settle_time) && (abs(x2_error) > error_band)
        is_done = double(1);
        fprintf('DEATH: settle timeout, err=%.3f after %.1fs (allowed=%.1fs)\n', ...
            abs(x2_error), next_time_since_change, allowed_settle_time);
        fprintf('\nx2=%.3f', x2)
    end

end

== matlab function Evaluation_RL_SMC_Env/Reward1 ==
  data: x1 input; x2 input; x2_ref input; u input; time_since_change input; v1 input; v2 input; reward output; x2_prev input; next_x2_prev output; u_prev input
function [reward, next_x2_prev] = calc_reward(x1, x2, x2_ref, u, time_since_change, v1, v2, x2_prev, u_prev)

% =========================================================================
% calc_reward.m — CMSD NN Controller Reward Function
%
% Argument order (must match Simulink block wiring):
%   x2, x2_ref, u, time_since_change, v1, v2, x2_prev, u_prev
%
% Key changes from previous version:
%   - violation^2 replaced with linear penalty  → fixes billion-reward bug
%   - per-step hard floor at -20                → agent always gets signal
%   - energy term scaled down (was dominating)  → u^2 → 0.01*(u/3500)^2
%   - v2 check uses abs(v2) (was unsigned)      → catches oscillation both ways
%   - all reward components kept proportional   → good ep ≈ +2000, bad ≈ -15000
% =========================================================================

% --- ENFORCE STRICT DATA TYPES FOR COMPILER ---
    reward       = double(0.1);
    next_x2_prev = double(x2);
    x2_error     = double(abs(x2_ref - x2));
    delta_u      = double(abs(u - u_prev));   % u is post-gain (Newtons)

% --- 1. TRACKING — primary goal (your original weights kept) ---
    reward = double(reward - (10.0 * x2_error^2));

% --- 2. TIGHT ZONE BONUS / MISS PENALTY ---
%   Your original ±1/+2 split kept, just clarified
    if x2_error < 0.01
        reward = double(reward + 2.0);    % inside 10mm — excellent
    elseif x2_error < 0.050
        reward = double(reward + 0.5);    % inside 50mm — acceptable
    else
        reward = double(reward - 1.0);    % outside — penalise
    end

% --- 3. SMC ROBUSTNESS — penalise oscillation after settling ---
%   abs(v2) catches oscillation in both directions (your version missed negative v2)
    if time_since_change > 1.0
        if abs(v2) > 0.01
            reward = double(reward - 5.0);
        end
    end

% --- 4. ENERGY EFFICIENCY ---
%   Scaled down from 0.5*(u/3500)^2 to 0.01*(u/3500)^2
%   Original was subtracting up to -0.5 per step just for moving — too aggressive
%   for early training where the agent NEEDS to move to explore.
%   At full force: 0.01 * 1^2 = -0.01 per step (negligible vs tracking signal)
    reward = double(reward - 0.01 * (u / 3500.0)^2);

% --- 5. HARDWARE LIMIT PENALTY — LINEAR, not squared ---
%   FIX: violation^2 was the billion-reward bug.
%   With gain=3500 and random actions, delta_u can reach 7000 N/step.
%   violation = 6500  →  violation^2 = 42,250,000 per step × 1500 steps = -63 billion.
%   Linear version: same signal to the agent (big jumps = bad) without explosion.
%   At worst case: -0.005 * 6500 = -32.5 per step — meaningful but survivable.
    if delta_u > 500.0
        violation = double(delta_u - 500.0);
        reward    = double(reward - (0.005 * violation));   % LINEAR — not squared
    end

% --- 6. VELOCITY DAMPING (your original weights kept) ---
    v1_penalty = double(abs(v1) * 0.02);
    v2_penalty = double(abs(v2) * 0.10);
    reward     = double(reward - v1_penalty - v2_penalty);

% --- 7. PER-STEP HARD FLOOR ---
%   Prevents any single catastrophic step from making the episode reward
%   so negative that the gradient update is meaningless noise.
%   Worst case episode: -20 * 1500 steps = -30,000  (was -2,315,943,825)
    reward = double(max(reward, -20.0));


        % --- THE ANTI-SUICIDE PATCH ---
    % If the AI violently jerks the motor and breaks the x1 limit, 
    % it receives a penalty so massive it will never do it again.
    if abs(x1) > 0.65
        reward = double(reward - 6000.0);
    end


end

== matlab function Evaluation_RL_SMC_Env/IsDone1 ==
  data: x1 input; is_done output; x2 input; x2_ref input; next_timer_03 output; timer_03 input; time_since_change input; current_step_size input; x2_ref_prev input; next_time_since_change output; next_step_size output; next_ref_prev output
function [is_done, next_timer_03, next_time_since_change, next_step_size, next_ref_prev] = check_safety(x1, x2, x2_ref, timer_03, time_since_change, current_step_size, x2_ref_prev)
    
    % --- ENFORCE STRICT DATA TYPES FOR THE COMPILER ---
    is_done = double(0); % <--- Changed to double(0) instead of false
    next_timer_03 = double(timer_03);
    next_time_since_change = double(time_since_change);
    next_step_size = double(current_step_size);
    next_ref_prev = double(x2_ref_prev);
    
    dt = double(0.01); 
    x2_error = double(x2_ref - x2);
    
    % --- 1. DETECT A REFERENCE CHANGE ---
    if abs(x2_ref - x2_ref_prev) > 0.001
        next_time_since_change = double(0.0);
        next_step_size = double(abs(x2_ref - x2_ref_prev));
    else
        next_time_since_change = double(time_since_change + dt);
    end
    next_ref_prev = double(x2_ref);
    
    % --- 2. DEATH CONDITIONS ---
    if abs(x1) > 0.65
        is_done = double(1); % <--- Changed to double(1) instead of true
    end
    
    if abs(x2_error) > 0.3
        next_timer_03 = double(timer_03 + dt);
    else
        next_timer_03 = double(0.0);
    end
    
    if next_timer_03 > 3.0 % <--- CHANGED TO 3.0 from 0.75
        is_done = double(1); % <--- Changed to double(1)
    end
    
    %if next_step_size > 0
    %    allowed_settle_time = double(next_step_size * 2.2);
    %else
    %    allowed_settle_time = double(2.0); 
    %end


    %=====> RELAXED: Give it a flat 5.0 seconds to settle, regardless of step size
    allowed_settle_time = double(5.0); % <--- BYPASS THE MULTIPLIER FOR NOW

    % Widen the survival boundary to 0.05m (50mm) for early training
    if (next_time_since_change > allowed_settle_time) && (abs(x2_error) > 0.050)
        is_done = double(1); % <--- Changed to double(1)
    end
end

== matlab function Evaluation_RL_SMC_Env/MATLAB Function ==
  data: x2_ref input; time_since_change output; x2_ref_prev input; time_since_change_prev input; next_x2_ref_prev output
function [time_since_change, next_x2_ref_prev] = time_since_change(x2_ref, x2_ref_prev, time_since_change_prev)
    
    % --- ENFORCE STRICT DATA TYPES ---
    dt = double(0.01); 
    time_since_change = double(0.0);
    next_x2_ref_prev  = double(x2_ref); % Always pass the current ref out for the next step
    
    % --- DETECT CHANGE ---
    x_ref_diff = double(abs(x2_ref - x2_ref_prev));
    
    if x_ref_diff >= 0.001
        % The target moved. Reset the stopwatch to zero.
        time_since_change = double(0.0);
    else
        % The target is stationary. Increment the stopwatch.
        time_since_change = double(time_since_change_prev + dt);
    end
    
end

== matlab function Evaluation_RL_SMC_Env/MATLAB Function1 ==
  data: u1 input; C2 output; u2 input; u3 input; u4 input; C4 output; Eta output; Phi output
function [C2, C4, Eta, Phi] = scale_actions(u1, u2, u3, u4)
    % =====================================================================
    % scale_actions.m
    % Converts the normalized [-1, 1] AI outputs into safe physical tuning 
    % boundaries for the Sliding Mode Controller.
    % =====================================================================

    % --- ENFORCE STRICT DATA TYPES ---
    u_1 = double(u1);
    u_2 = double(u2);
    u_3 = double(u3);
    u_4 = double(u4);

    % --- 1. C2: Speed vs. Overshoot ---
    % Baseline: 20.0 | Ceiling: 25.0 | Safe Range: [15.0 to 25.0]
    % If u1 = 1, C2 = 25. If u1 = -1, C2 = 15.
    C2 = double(20.0 + (5.0 * u_1));

    % --- 2. C4: Damping ---
    % Baseline: 2.0 | Scale: 1.0 | Safe Range: [1.0 to 3.0]
    C4 = double(2.0 + (1.0 * u_2));

    % --- 3. Eta: Reaching Law (Steady-State Error) ---
    % Center: 100.0 | Scale: 50.0 | Safe Range: [50.0 to 150.0]
    Eta = double(100.0 + (50.0 * u_3));

    % --- 4. Phi: Boundary Layer (Chatter Killer) ---
    % Center: 0.100 | Scale: 0.070 | Safe Range: [0.030 to 0.170]
    % Ensures Phi never drops below the 0.027 chatter threshold.
    Phi = double(0.100 + (0.070 * u_4));
end

== matlab function Evaluation_RL_SMC_Env/Reward2 ==
  data: x1 input; x2 input; x2_ref input; u input; time_since_change input; v1 input; v2 input; reward output; next_u_prev output; u_prev input
function [reward, next_u_prev] = calc_reward(x1, x2, x2_ref, u, time_since_change, v1, v2, u_prev)

% =========================================================================
% calc_reward.m — Phase 1: 50Hz Bounded Slalom
% Focus: Smooth tracking, scaled continuous rewards.
% =========================================================================

% --- ENFORCE STRICT DATA TYPES ---
    reward       = double(0.2);           % Scaled base survival
    next_u_prev  = double(u);             
    x2_error     = double(abs(x2_ref - x2));
    delta_u      = double(abs(u - u_prev));
    x1_abs       = double(abs(x1));

% --- 1. TRACKING (RISE TIME AGGRESSION) ---
    reward = double(reward - (4.0 * x2_error^2));

% --- 2. FORGIVING PARACHUTE (50mm warning zone) ---
    if (x2_error < 0.050) && (abs(v2) > 0.10)
        reward = double(reward - (1.0 * abs(v2)));
    end

% --- 3. TARGET LOCK BONUS ---
    if x2_error < 0.010
        reward = double(reward + 0.6);    % inside 10mm 
    elseif x2_error < 0.030
        reward = double(reward + 0.3);    % inside 30mm (Matches Settle Boundary)
    end

% --- 4. CONTINUOUS PROGRESS BONUS ---
    progress_bonus = double(0.2 * exp(-5.0 * x2_error^2));
    reward = double(reward + progress_bonus);

% --- 5. CHATTER REDUCTION (SMOOTH THE SMC) ---
    if delta_u > 50.0
        reward = double(reward - (0.002 * delta_u));
    end

% --- 6. X1 SOFT BARRIER & CENTERING ---
    if x1_abs > 0.30
        x1_margin1 = double(x1_abs - 0.30);
        reward = double(reward - (1.6 * x1_margin1^2));
    end
    x1_centre_bonus = double(0.06 * exp(-10.0 * x1^2));
    reward = double(reward + x1_centre_bonus);

% --- 7. TERMINAL PENALTY ---
    if x1_abs > 0.65
        reward = double(reward - 200.0);
    end

% --- 8. PER-STEP HARD FLOOR ---
    reward = double(max(reward, -10.0));

end

== matlab function Evaluation_RL_SMC_Env/IsDone2 ==
  data: x1 input; is_done output; x2 input; x2_ref input; next_timer_03 output; timer_03 input; time_since_change input; current_step_size input; x2_ref_prev input; next_time_since_change output; next_step_size output; next_ref_prev output
function [is_done, next_timer_03, next_time_since_change, next_step_size, next_ref_prev] = check_safety(x1, x2, x2_ref, timer_03, time_since_change, current_step_size, x2_ref_prev)

% =========================================================================
% check_safety.m — Phase 1: 50Hz Bounded Slalom
% Focus: 2.5s Settle-Time & Hardware Protection
% =========================================================================

% --- ENFORCE STRICT DATA TYPES ---
    is_done                = double(0);
    next_timer_03          = double(timer_03);
    next_time_since_change = double(time_since_change);
    next_step_size         = double(current_step_size);
    next_ref_prev          = double(x2_ref_prev);
    
    dt       = double(0.02); % 50Hz AI clock 
    x2_error = double(x2_ref - x2);

% --- 1. REFERENCE CHANGE DETECTION ---
    if abs(x2_ref - x2_ref_prev) > 0.001
        next_time_since_change = double(0.0);
        next_step_size         = double(abs(x2_ref - x2_ref_prev));
    else
        next_time_since_change = double(time_since_change + dt);
    end
    next_ref_prev = double(x2_ref);

% --- 2. DEATH A: Hardware Limit (x1 wall) ---
    if abs(x1) > 0.65
        is_done = double(1);
    end

% --- 3. DEATH B: Total Loss of Control ---
    if abs(x2_error) > 0.5
        next_timer_03 = double(timer_03 + dt);
    else
        next_timer_03 = double(0.0);
    end
    
    if next_timer_03 > 3.0
        is_done = double(1);
    end

% --- 4. DEATH C: The Slalom Settle-Time ---
% Because the jump happens every 3.0s, give it 2.5s to settle.
    allowed_settle_time = double(2.5);
    error_band          = double(0.030); % Forgiving 30mm boundary
    
    if (next_time_since_change > allowed_settle_time) && (abs(x2_error) > error_band)
        is_done = double(1);
    end

end
